simulink model "MATE_SwitchedReluctanceMotor64Drive"  (R2024b)
settings: Solver=FixedStepDiscrete  StartTime=0.0  StopTime=5  FixedStep=Ts  RelTol=1e-3  AbsTol=1e-5  EnableMultiTasking=on
PreLoadFcn:
  | Ts=1e-6;Rsnu=100; Csnu=1e-6;
  | 
  | % Magnetisation characteristic table of the switched Reluctance Motor:
  | % Table elements =  Flux linkage, in Wb.
  | 
  | FluxTable = [
  |     0             0              0             0             0             0
  |     0.3220    0.3050    0.2280    0.1240    0.0220    0.0170
  |     0.3760    0.3570    0.2770    0.1600    0.0420    0.0340
  |     0.3990    0.3850    0.3000    0.1830    0.0640    0.0500
  |     0.4160    0.4020    0.3200    0.2010    0.0840    0.0670
  |     0.4280    0.4150    0.3340    0.2190    0.1030    0.0840
  |     0.4370    0.4260    0.3480    0.2370    0.1230    0.1010
  |     0.4430    0.4330    0.3590    0.2530    0.1420    0.1170
  |     0.4490    0.4390    0.3710    0.2680    0.1610    0.1340
  |     0.4540    0.4440    0.3820    0.2820    0.1790    0.1510
  |     0.4590    0.4490    0.3920    0.2950    0.1970    0.1680
  |     0.4630    0.4530    0.4020    0.3090    0.2140    0.1840
  |     0.4670    0.4570    0.4110    0.3220    0.2310    0.2010
  |     0.4700    0.4620    0.4190    0.3360    0.2460    0.2180
  |     0.4740    0.4650    0.4270    0.3480    0.2610    0.2350
  |     0.4780    0.4690    0.4330    0.3590    0.2770    0.2510
  |     0.4810    0.4730    0.4380    0.3690    0.2910    0.2680
  |     0.4840    0.4770    0.4440    0.3800    0.3050    0.2850
  |     0.4870    0.4790    0.4480    0.3890    0.3200    0.3020];
  | 
  | % Table columns :  Rotor angles, in degrees.
  | 
  | RotorAngles = [
  |     0             10            20            30            40            45];
  | 
  | % Table rows : Stator current, in A.
  | 
  | StatorCurrents = [ 0:size(FluxTable,1)-1] * 25;
PostLoadFcn:
  | Ts=1e-6;Rsnu=100; Csnu=1e-6;
  | 
  | % Magnetisation characteristic table of the switched Reluctance Motor:
  | % Table elements =  Flux linkage, in Wb.
  | 
  | FluxTable = [
  |     0             0              0             0             0             0
  |     0.3220    0.3050    0.2280    0.1240    0.0220    0.0170
  |     0.3760    0.3570    0.2770    0.1600    0.0420    0.0340
  |     0.3990    0.3850    0.3000    0.1830    0.0640    0.0500
  |     0.4160    0.4020    0.3200    0.2010    0.0840    0.0670
  |     0.4280    0.4150    0.3340    0.2190    0.1030    0.0840
  |     0.4370    0.4260    0.3480    0.2370    0.1230    0.1010
  |     0.4430    0.4330    0.3590    0.2530    0.1420    0.1170
  |     0.4490    0.4390    0.3710    0.2680    0.1610    0.1340
  |     0.4540    0.4440    0.3820    0.2820    0.1790    0.1510
  |     0.4590    0.4490    0.3920    0.2950    0.1970    0.1680
  |     0.4630    0.4530    0.4020    0.3090    0.2140    0.1840
  |     0.4670    0.4570    0.4110    0.3220    0.2310    0.2010
  |     0.4700    0.4620    0.4190    0.3360    0.2460    0.2180
  |     0.4740    0.4650    0.4270    0.3480    0.2610    0.2350
  |     0.4780    0.4690    0.4330    0.3590    0.2770    0.2510
  |     0.4810    0.4730    0.4380    0.3690    0.2910    0.2680
  |     0.4840    0.4770    0.4440    0.3800    0.3050    0.2850
  |     0.4870    0.4790    0.4480    0.3890    0.3200    0.3020];
  | 
  | % Table columns :  Rotor angles, in degrees.
  | 
  | RotorAngles = [
  |     0             10            20            30            40            45];
  | 
  | % Table rows : Stator current, in A.
  | 
  | StatorCurrents = [ 0:size(FluxTable,1)-1] * 25;
InitFcn:
  | Ts=1e-6;Rsnu=100; Csnu=1e-6;
  | 
  | % Magnetisation characteristic table of the switched Reluctance Motor:
  | % Table elements =  Flux linkage, in Wb.
  | 
  | FluxTable = [
  |     0             0              0             0             0             0
  |     0.3220    0.3050    0.2280    0.1240    0.0220    0.0170
  |     0.3760    0.3570    0.2770    0.1600    0.0420    0.0340
  |     0.3990    0.3850    0.3000    0.1830    0.0640    0.0500
  |     0.4160    0.4020    0.3200    0.2010    0.0840    0.0670
  |     0.4280    0.4150    0.3340    0.2190    0.1030    0.0840
  |     0.4370    0.4260    0.3480    0.2370    0.1230    0.1010
  |     0.4430    0.4330    0.3590    0.2530    0.1420    0.1170
  |     0.4490    0.4390    0.3710    0.2680    0.1610    0.1340
  |     0.4540    0.4440    0.3820    0.2820    0.1790    0.1510
  |     0.4590    0.4490    0.3920    0.2950    0.1970    0.1680
  |     0.4630    0.4530    0.4020    0.3090    0.2140    0.1840
  |     0.4670    0.4570    0.4110    0.3220    0.2310    0.2010
  |     0.4700    0.4620    0.4190    0.3360    0.2460    0.2180
  |     0.4740    0.4650    0.4270    0.3480    0.2610    0.2350
  |     0.4780    0.4690    0.4330    0.3590    0.2770    0.2510
  |     0.4810    0.4730    0.4380    0.3690    0.2910    0.2680
  |     0.4840    0.4770    0.4440    0.3800    0.3050    0.2850
  |     0.4870    0.4790    0.4480    0.3890    0.3200    0.3020];
  | 
  | % Table columns :  Rotor angles, in degrees.
  | 
  | RotorAngles = [
  |     0             10            20            30            40            45];
  | 
  | % Table rows : Stator current, in A.
  | 
  | StatorCurrents = [ 0:size(FluxTable,1)-1] * 25;
undefined symbols (not defined in the file or in its folder): DiscIntNeverNeededParam
libraries: ee_lib x12, nesl_utility x10, fl_lib x6, simetranss x5
(part 2 of 2)

== system MATE_SwitchedReluctanceMotor64Drive/Validation drive  only/Three-arm bridge/IGBT5 ==
  G : Inport
  IGBT : ee_lib/Semiconductors & Converters/IGBT (Ideal, Switching)  port_option=ee.enum.controlport.ps  Vf=0.1 V  Ron=0.01 Ohm  Goff=1e-5 1/Ohm  Vth=0.5 V  diode_param=ee.enum.semiconductors.protectionDiode.external  diode_Vf=0.6 V  diode_Ron=0.03 Ohm  diode_Goff=1e-5 1/Ohm  diode_C=5e-8 F  diode_iRM=-235 A  diode_iF=300 A  diode_idot=-50 A/us  diode_trr_param=1  diode_trr_factor=3  diode_trr=15 us  diode_Qrr=1.5e+3 s*uA  ice_specify=off  ice_priority=None  ice=0 A  ice_nominal_specify=off  ice_nominal_value=1  ice_nominal_unit=A  vce_specify=off  vce_priority=None  vce=0 V  vce_nominal_specify=off  vce_nominal_value=1  vce_nominal_unit=V  vge_specify=off  vge_priority=None  vge=0 V  vge_nominal_specify=off  vge_nominal_value=1  vge_nominal_unit=V  thermal_loss_option=ee.enum.converters.thermalLossOption.constantvalues  Von_data=[0, .1, .6, .8, 1, 1.3, 1.6, 2, 2.4; 0, .1, .7, 1, 1.2, 1.5, 1.9, 2.4, 2.8] V  Tj=[298.15, 398.15] K  Iout_data=[0, .1, 1, 5, 10, 20, 40, 70, 100] A  Eon_data=[0, .0024, .024, .12, .2, .48, 1.04, 2.16, 3.24; 0, .003, .03, .15, .25, .6, 1.3, 2.7, 4.05] * 1e-3 J  Eoff_data=[0, .0007, .0066, .033, .066, .17, .33, .83, 1.5; 0, .001, .01, .05, .1, .25, .5, 1.2, 2.2] * 1e-3 J  Eon_data_3D=[zeros(2, 9, 3)] J  Eoff_data_3D=[zeros(2, 9, 3)] J  Tj_loss=[298.15, 398.15] K  Iout_data_loss=[0, .1, 1, 5, 10, 20, 40, 70, 100] A  tabulateWithVce=false  Vce_loss=[0, 150, 300] V  Eon_scalar=22.86e-3 J  Eoff_scalar=17.14e-3 J  Voff=300 V  Iout_scalar=600 A  useCurrentFromPreviousCycle=false  useVoltageFromPreviousCycle=false  diodeModelType=ee.enum.converters.diodeModelType.pwl  diodeTableType=ee.enum.diode.tableType.IfMat  diode_ReverseIVType=ee.enum.diode.diodeReverseIV.constant  diode_IfMat=[.07, .12, .19, 1.75, 4.24, 7.32, 11.2; .16, .3, .72, 2.14, 4.02, 6.35, 9.12] A  diode_VfMat=[.9, 1.15, 1.25, 1.5, 1.75, 2.17, 2.6, 2.85; .58, .68, .75, 1.1, 1.38, 1.77, 2.27, 2.7] V  diode_TjVec=[25, 125] degC  diode_VfVec=[.5, .7, .9, 1.3, 1.7, 2.1, 2.5] V  diode_IfVec=[.1, .2, .5, 1, 2, 4, 7, 10] A  diode_IrMat=[1e-06, 2e-06, 5e-06, 1e-05, 2.5e-05, 5e-05, .0001; 2e-06, 5e-06, 1e-05, 4e-05, 8e-05, .0002, .0005] A  diode_VrMat=[10, 100, 200, 250, 300, 325, 350; 10, 70, 160, 220, 270, 300, 320] V  diode_VrVec=[10, 20, 40, 50, 70, 80, 100] V  diode_IrVec=[1e-06, 2e-06, 5e-06, 1e-05, 2e-05, 5e-05, .0001] A  diode_Vr=-600 V  diode_Ls=150 nH  diode_Erec=0.03 J  diode_rec_loss_model=ee.enum.diode.reverseRecoveryModel.fixed  diode_ErecVal=0 J  diode_scaleWithIandV=true  diode_ErecMat=zeros(2, 3) J  diode_TjrecVec=[298.15, 398.15] K  diode_IfrecVec=[.1, 1, 10] A  diode_IrecVal=10 A  diode_VrecVal=10 V  diode_tFilter=1 / 1000 / 100 s  separateThermalPortForDiode=false  thermal_network_parameterization=ee.enum.thermalNetworkTopology.external  Rth=[.08, .5] K/W  Rth_Cauer=[.08, .1, .5] K/W  Rth_Foster=[.08, .14, .22, .16] K/W  thermal_mass_parameterization=ee.enum.thermalNetwork.timeconstant  thermal_mass=[.01, .5] J/K  thermal_mass_Cauer=[.01, .1, .5] J/K  thermal_mass_Foster=[.001, .005, .05, .5] J/K  thermal_time_constant=[.001, .2] s  thermal_time_constant_Cauer=[.001, .1, .2] s  thermal_time_constant_Foster=[7e-05, .0007, .01, .08] s  thermal_mass_initial_temperatures=[25, 25] degC  thermal_mass_initial_temperatures_Cauer=[25, 25, 25] degC  junction_thermal_mass=0.01 J/K  Tvec_initial_Foster=[25, 25, 25, 25] degC  RthDiode=[.03, .2] K/W  RthCauerDiode=[.03, .1, .2] K/W  RthFosterDiode=[.03, .2] K/W  thermalMassDiode=[3, 25] J/K  thermalMassCauerDiode=[3, 10, 25] J/K  thermalMassFosterDiode=[33, 50] J/K  thermalTauDiode=[.1, 5] s  thermalTauCauerDiode=[.1, 1, 5] s  thermalTauFosterDiode=[1, 10] s  thermalMassInitTempDiode=[25, 25] degC  thermalMassInitTempCauerDiode=[25, 25, 25] degC  junctionthermalMassDiode=0.1 J/K  TVecInitialFosterDiode=[25, 25, 25, 25] degC  no_thermal_network=0  IGBT_junction_temperature_specify=off  IGBT_junction_temperature_priority=None  IGBT_junction_temperature=25 degC  IGBT_junction_temperature_nominal_specify=off  IGBT_junction_temperature_nominal_value=1  IGBT_junction_temperature_nominal_unit=degC  diode_junction_temperature_specify=off  diode_junction_temperature_priority=None  diode_junction_temperature=25 degC  diode_junction_temperature_nominal_specify=off  diode_junction_temperature_nominal_value=1  diode_junction_temperature_nominal_unit=degC  Qj_specify=off  Qj_priority=None  Qj=0 W  Qj_nominal_specify=off  Qj_nominal_value=1  Qj_nominal_unit=W  accumulatedSwitchingLosses_specify=off  accumulatedSwitchingLosses_priority=None  accumulatedSwitchingLosses=0 J
  Simulink-PS Converter : nesl_utility/Simulink-PS Converter  PhysicalDomain=network_engine_domain  SubClassName=ps_input  LeftPortType=input  RightPortType=output  PseudoPeriodic=off  Frequencies=[]  NoiseDistribution=none  NoiseParameters=[]  Unit=V  AffineConversion=off  FilteringAndDerivatives=zero  SimscapeFilterOrder=1  InputFilterTimeConstant=.001  UdotUserProvided=1
  C : PMIOPort  Side=Right
  E : PMIOPort  Port=2  Side=Right
  wires:
  G/1 -> Simulink-PS Converter/1
  connections:
  Simulink-PS Converter/RConn1 -- IGBT/LConn1
  IGBT/RConn2 -- E/RConn1
  IGBT/RConn1 -- C/RConn1

== system MATE_SwitchedReluctanceMotor64Drive/Validation drive  only/Three-arm bridge/IGBT6 ==
  G : Inport
  IGBT : ee_lib/Semiconductors & Converters/IGBT (Ideal, Switching)  port_option=ee.enum.controlport.ps  Vf=0.1 V  Ron=0.01 Ohm  Goff=1e-5 1/Ohm  Vth=0.5 V  diode_param=ee.enum.semiconductors.protectionDiode.external  diode_Vf=0.6 V  diode_Ron=0.03 Ohm  diode_Goff=1e-5 1/Ohm  diode_C=5e-8 F  diode_iRM=-235 A  diode_iF=300 A  diode_idot=-50 A/us  diode_trr_param=1  diode_trr_factor=3  diode_trr=15 us  diode_Qrr=1.5e+3 s*uA  ice_specify=off  ice_priority=None  ice=0 A  ice_nominal_specify=off  ice_nominal_value=1  ice_nominal_unit=A  vce_specify=off  vce_priority=None  vce=0 V  vce_nominal_specify=off  vce_nominal_value=1  vce_nominal_unit=V  vge_specify=off  vge_priority=None  vge=0 V  vge_nominal_specify=off  vge_nominal_value=1  vge_nominal_unit=V  thermal_loss_option=ee.enum.converters.thermalLossOption.constantvalues  Von_data=[0, .1, .6, .8, 1, 1.3, 1.6, 2, 2.4; 0, .1, .7, 1, 1.2, 1.5, 1.9, 2.4, 2.8] V  Tj=[298.15, 398.15] K  Iout_data=[0, .1, 1, 5, 10, 20, 40, 70, 100] A  Eon_data=[0, .0024, .024, .12, .2, .48, 1.04, 2.16, 3.24; 0, .003, .03, .15, .25, .6, 1.3, 2.7, 4.05] * 1e-3 J  Eoff_data=[0, .0007, .0066, .033, .066, .17, .33, .83, 1.5; 0, .001, .01, .05, .1, .25, .5, 1.2, 2.2] * 1e-3 J  Eon_data_3D=[zeros(2, 9, 3)] J  Eoff_data_3D=[zeros(2, 9, 3)] J  Tj_loss=[298.15, 398.15] K  Iout_data_loss=[0, .1, 1, 5, 10, 20, 40, 70, 100] A  tabulateWithVce=false  Vce_loss=[0, 150, 300] V  Eon_scalar=22.86e-3 J  Eoff_scalar=17.14e-3 J  Voff=300 V  Iout_scalar=600 A  useCurrentFromPreviousCycle=false  useVoltageFromPreviousCycle=false  diodeModelType=ee.enum.converters.diodeModelType.pwl  diodeTableType=ee.enum.diode.tableType.IfMat  diode_ReverseIVType=ee.enum.diode.diodeReverseIV.constant  diode_IfMat=[.07, .12, .19, 1.75, 4.24, 7.32, 11.2; .16, .3, .72, 2.14, 4.02, 6.35, 9.12] A  diode_VfMat=[.9, 1.15, 1.25, 1.5, 1.75, 2.17, 2.6, 2.85; .58, .68, .75, 1.1, 1.38, 1.77, 2.27, 2.7] V  diode_TjVec=[25, 125] degC  diode_VfVec=[.5, .7, .9, 1.3, 1.7, 2.1, 2.5] V  diode_IfVec=[.1, .2, .5, 1, 2, 4, 7, 10] A  diode_IrMat=[1e-06, 2e-06, 5e-06, 1e-05, 2.5e-05, 5e-05, .0001; 2e-06, 5e-06, 1e-05, 4e-05, 8e-05, .0002, .0005] A  diode_VrMat=[10, 100, 200, 250, 300, 325, 350; 10, 70, 160, 220, 270, 300, 320] V  diode_VrVec=[10, 20, 40, 50, 70, 80, 100] V  diode_IrVec=[1e-06, 2e-06, 5e-06, 1e-05, 2e-05, 5e-05, .0001] A  diode_Vr=-600 V  diode_Ls=150 nH  diode_Erec=0.03 J  diode_rec_loss_model=ee.enum.diode.reverseRecoveryModel.fixed  diode_ErecVal=0 J  diode_scaleWithIandV=true  diode_ErecMat=zeros(2, 3) J  diode_TjrecVec=[298.15, 398.15] K  diode_IfrecVec=[.1, 1, 10] A  diode_IrecVal=10 A  diode_VrecVal=10 V  diode_tFilter=1 / 1000 / 100 s  separateThermalPortForDiode=false  thermal_network_parameterization=ee.enum.thermalNetworkTopology.external  Rth=[.08, .5] K/W  Rth_Cauer=[.08, .1, .5] K/W  Rth_Foster=[.08, .14, .22, .16] K/W  thermal_mass_parameterization=ee.enum.thermalNetwork.timeconstant  thermal_mass=[.01, .5] J/K  thermal_mass_Cauer=[.01, .1, .5] J/K  thermal_mass_Foster=[.001, .005, .05, .5] J/K  thermal_time_constant=[.001, .2] s  thermal_time_constant_Cauer=[.001, .1, .2] s  thermal_time_constant_Foster=[7e-05, .0007, .01, .08] s  thermal_mass_initial_temperatures=[25, 25] degC  thermal_mass_initial_temperatures_Cauer=[25, 25, 25] degC  junction_thermal_mass=0.01 J/K  Tvec_initial_Foster=[25, 25, 25, 25] degC  RthDiode=[.03, .2] K/W  RthCauerDiode=[.03, .1, .2] K/W  RthFosterDiode=[.03, .2] K/W  thermalMassDiode=[3, 25] J/K  thermalMassCauerDiode=[3, 10, 25] J/K  thermalMassFosterDiode=[33, 50] J/K  thermalTauDiode=[.1, 5] s  thermalTauCauerDiode=[.1, 1, 5] s  thermalTauFosterDiode=[1, 10] s  thermalMassInitTempDiode=[25, 25] degC  thermalMassInitTempCauerDiode=[25, 25, 25] degC  junctionthermalMassDiode=0.1 J/K  TVecInitialFosterDiode=[25, 25, 25, 25] degC  no_thermal_network=0  IGBT_junction_temperature_specify=off  IGBT_junction_temperature_priority=None  IGBT_junction_temperature=25 degC  IGBT_junction_temperature_nominal_specify=off  IGBT_junction_temperature_nominal_value=1  IGBT_junction_temperature_nominal_unit=degC  diode_junction_temperature_specify=off  diode_junction_temperature_priority=None  diode_junction_temperature=25 degC  diode_junction_temperature_nominal_specify=off  diode_junction_temperature_nominal_value=1  diode_junction_temperature_nominal_unit=degC  Qj_specify=off  Qj_priority=None  Qj=0 W  Qj_nominal_specify=off  Qj_nominal_value=1  Qj_nominal_unit=W  accumulatedSwitchingLosses_specify=off  accumulatedSwitchingLosses_priority=None  accumulatedSwitchingLosses=0 J
  Simulink-PS Converter : nesl_utility/Simulink-PS Converter  PhysicalDomain=network_engine_domain  SubClassName=ps_input  LeftPortType=input  RightPortType=output  PseudoPeriodic=off  Frequencies=[]  NoiseDistribution=none  NoiseParameters=[]  Unit=V  AffineConversion=off  FilteringAndDerivatives=zero  SimscapeFilterOrder=1  InputFilterTimeConstant=.001  UdotUserProvided=1
  C : PMIOPort  Side=Right
  E : PMIOPort  Port=2  Side=Right
  wires:
  G/1 -> Simulink-PS Converter/1
  connections:
  IGBT/RConn1 -- C/RConn1
  IGBT/RConn2 -- E/RConn1
  Simulink-PS Converter/RConn1 -- IGBT/LConn1
